simulink model "tb_rc_link_speed"  (R2026b)
values from neighbouring files (symbols this model uses):
  P = tc.P; P.rc.p_loss = 0    [t_rc_link.m]    (also in t_row_driver.m = shaddad_params('Assign', false); t_row_test_system.m = t_row_test_system.vcValue(res, 'P'))
  Ts = prm.Ts    [row_driver_bench.m]
settings Model: Creator=aomar  LastModifiedBy=aomar

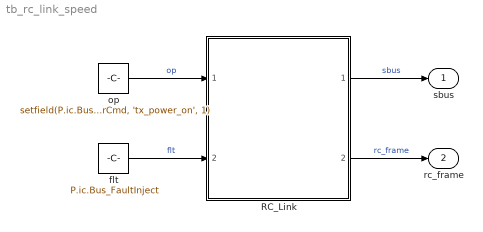
== system tb_rc_link_speed ==
  RC_Link : Subsystem  ReferencedSubsystem=RC_Link_Sim
  flt : Constant  Value=P.ic.Bus_FaultInject  OutDataTypeStr=Bus: Bus_FaultInject  SampleTime=Ts.ctrl
  op : Constant  Value=setfield(P.ic.Bus_OperatorCmd, 'tx_power_on', 1)  OutDataTypeStr=Bus: Bus_OperatorCmd  SampleTime=Ts.ctrl
  sbus : Outport  OutDataTypeStr=Bus: Bus_SbusStream
  rc_frame : Outport  Port=2  OutDataTypeStr=Bus: Bus_RcFrame
  wires:
  op/1 -> RC_Link/1  "op"
  flt/1 -> RC_Link/2  "flt"
  RC_Link/1 -> sbus/1  "sbus"
  RC_Link/2 -> rc_frame/1  "rc_frame"
